simulink model "traj_rigid_body_example"  (R2018b)
settings: Solver=ode2  StartTime=0.0  StopTime=60  FixedStep=0.001  RelTol=1e-3
values from neighbouring files (symbols this model uses):
  cycle = true    [traj_controller_mass_point_example_init.m]    (also in traj_from_waypoints_example.m = false; traj_rigid_body_example_init.m)
  g = 9.81    [traj_controller_mass_point_example_init.m]    (also in traj_from_waypoints_example.m; traj_rigid_body_example_init.m)
  inital_point = waypoints(:,1)    [traj_controller_mass_point_example_init.m]    (also in traj_rigid_body_example_init.m)
  inital_vel_vec = inital_velo * T    [traj_controller_mass_point_example_init.m]    (also in traj_rigid_body_example_init.m)
  traj = trajFromWaypoints(traj_empty, waypoints, degree, cycle)    [traj_controller_mass_point_example_init.m]    (also in traj_from_waypoints_example.m = trajFromWaypoints(traj, waypoints, degree, cycle); traj_rigid_body_example_init.m)
  waypoints = [1 -1 0.2; 2 0 0.1; 1 1 0; -1 -1 0; -2 0 0.1; -1 1 0.2]'*50    [traj_controller_mass_point_example_init.m]    (also in traj_from_waypoints_example.m = [1 1 1; 2 2 2; 3 3 3; 4 4 4]'; traj_rigid_body_example_init.m)
libraries: actuators_lib x8, traj_lib x3, axes_transformation_lib x3, flightgear_visualization_lib x1, sensors_lib x1, quatAttitudeController_lib x1, rigidBody_lib x1
settings Model: Creator=Fgücker  LastModifiedBy=yannic

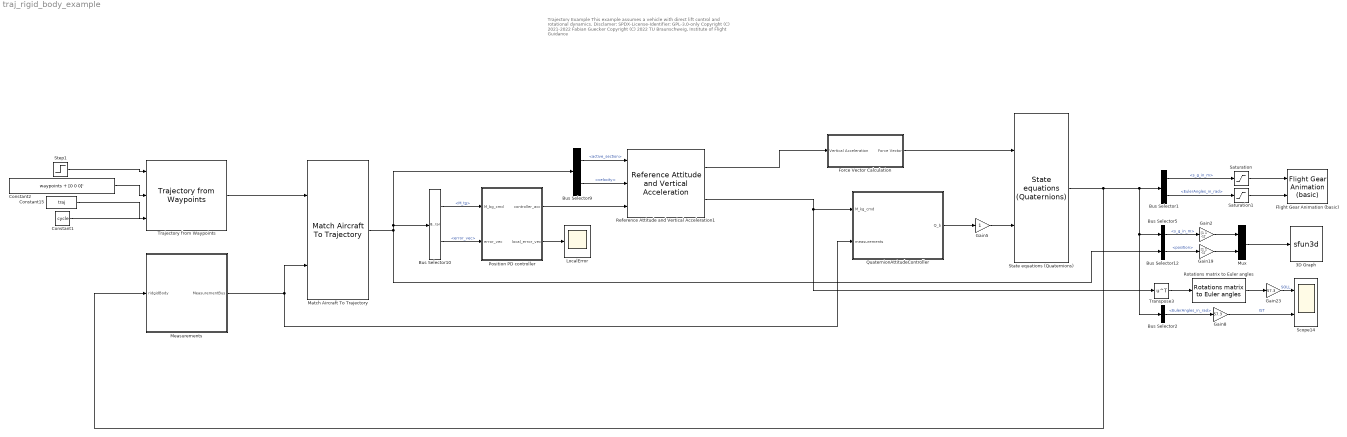
== system traj_rigid_body_example ==
  note: Trajectory Example
      |
      | This example assumes a vehicle with direct lift control and rotational dynamics.
      |
      | Disclamer:
      | SPDX-License-Identifier: GPL-3.0-only
      |
      | Copyright (C) 2021-2022 Fabian Guecker
      | Copyright (C) 2022 TU Braunschweig, Institute of Flight Guidance
  3D Graph : S-Function  LoadFcn=if exist('sfun3d','file'), sfun3d([],[],[],'LoadBlock'); end  FunctionName=sfun3d  Parameters=ax,T,np,cp,gd,ls,mk,mx,hd,tb  SFunctionDeploymentMode=off  EnableBusSupport=off  mask(3D Graph){np=2, ax=[-8 8 -8 8 -8 8]*20, mx=1e4, T=0.040, cp=[-1 -1 1]*50, gd=on, hd=off, tb=off, ls=-, mk=none}
      mask prompts: np "Number of moving points (lines)"; ax "Range: [xmin xmax  ymin ymax zmin zmax]"; mx "Max number of points in each line"; T "Sampling Time"; cp "Camera position (use [0 0 1] for 2D XY view)"; gd "Grid (on|off)"; hd "HeadMarkers (on|off)"; tb "Toolbar (on|off)"; ls "LineStyle"; mk "LineMarker"
      mask help:
      | This block plots the position of several points in the XYZ space. The input contains the coordinates of all the points (x1,y1,z1,x2,y2,z2,...).
      | The number of moving points (lines), the XYZ ranges, sampling time, camera position, and grid (among other things) can be set as mask parameters.
      settings: CopyFcn=if exist('sfun3d','file'), sfun3d([],[],[],'CopyBlock'); end  DeleteFcn=if exist('sfun3d','file'), sfun3d([],[],[],'DeleteBlock'); end  NameChangeFcn=if exist('sfun3d','file'), sfun3d([],[],[],'NameChange'); end
      mask Help:
      | This block plots the position of several points in the XYZ space. The input contains the coordinates of all the points (x1,y1,z1,x2,y2,z2,...).
      | The number of moving points (lines), the XYZ ranges, sampling time, camera position, and grid (among other things) can be set as mask parameters.
      mask TypeOptions ls: - | -- | : | -. | none
      mask TypeOptions mk: none | . | + | o | * | x | square | diamond | v | ^ | > | < | pentagram | hexagram
      mask Display: plot([.05 .95 .95 .05 .05],[.45 .45 .95 .95 .45], 0.5+cos(0:0.1:2*pi)*0.3,0.7+sin(0:0.1:2*pi)*0.2)
  Bus Selector1 : BusSelector  OutputSignals=s_g_in_m,EulerAngles_in_rad
  Bus Selector10 : BusSelector  OutputSignals=M_tg,error_vec
  Bus Selector12 : BusSelector  OutputSignals=position
  Bus Selector2 : BusSelector  OutputSignals=EulerAngles_in_rad
  Bus Selector5 : BusSelector  OutputSignals=s_g_in_m
  Bus Selector9 : BusSelector  OutputSignals=active_section,velocity
  Constant1 : Constant  Value=cycle  OutDataTypeStr=boolean
  Constant15 : Constant  Value=traj  OutDataTypeStr=Bus: trajectoryBus
  Constant2 : Constant  Value=waypoints + [0 0 0]'
  Flight Gear Animation (basic) : flightgear_visualization_lib/Flight Gear Animation (basic)  inital_lat=63.985024  inital_long=-22.597652  inital_height=70  remoteURL='127.0.0.1'  remotePort=5502
      settings: SourceProductName=LADAC
  Force Vector Calculation : Subsystem  mask{m=1}
      mask prompts: m "Mass of the aircraft"
  Gain19 : Gain  Gain=[1 1 -1]'
  Gain2 : Gain  Gain=[1 1 -1]'
  Gain23 : Gain  Gain=57.3
  Gain5 : Gain
  Gain8 : Gain  Gain=57.3
  LocalError : Scope
  Match Aircraft To Trajectory : traj_lib/Match Aircraft To Trajectory
      settings: SourceProductName=LADAC
  Measurements : Subsystem  mask{omega0=100, D=1}
      mask prompts: omega0 "Omega - Filter"; D "Damping D - Filter"
  Mux : Mux  Inputs=2
  Position PD controller : Subsystem
  QuaternionAttitudeController : Subsystem
  Reference Attitude and Vertical Acceleration1 : traj_lib/Reference Attitude and Vertical Acceleration  G0=9.81
      settings: SourceProductName=LADAC
  Rotations matrix to Euler angles : axes_transformation_lib/Rotations matrix to Euler angles  SystemSampleTime=-1
      settings: SourceProductName=LADAC
  Saturation : Saturate  UpperLimit=5000  LowerLimit=-5000
  Saturation1 : Saturate  UpperLimit=100*pi  LowerLimit=-100*pi
  Scope14 : Scope  NumInputPorts=2
  State equations (Quaternions) : rigidBody_lib/State equations (Quaternions)  m=1  I=eye(3)  g=9.81  omega_Kb_0=[0,0,0]'  q_bg_0=inital_quaternion'  V_Kb_0=[norm(inital_vel_vec);0;0]  s_g_0=inital_point+[0 0 0]'
  Step1 : Step  Time=0  SampleTime=0
  Trajectory from Waypoints : traj_lib/Trajectory from Waypoints  traj_params=traj_params
      settings: SourceProductName=LADAC
  Transpose3 : Math  Operator=transpose  SaturateOnIntegerOverflow=on
  wires:
  Bus Selector1/2 -> Saturation1/1  "<EulerAngles_in_rad>"
  Bus Selector1/1 -> Saturation/1  "<s_g_in_m>"
  QuaternionAttitudeController/1(Q_b) -> Gain5/1
  Bus Selector2/1 -> Gain8/1  "<EulerAngles_in_rad>"
  Bus Selector5/1 -> Gain2/1  "<s_g_in_m>"
  State equations (Quaternions)/1 -> Measurements/1(ridgidBody), Bus Selector5/1, Bus Selector2/1, Bus Selector1/1
  Saturation/1 -> Flight Gear Animation (basic)/1
  Saturation1/1 -> Flight Gear Animation (basic)/2
  Gain5/1 -> State equations (Quaternions)/2
  Gain2/1 -> Mux/1
  Mux/1 -> 3D Graph/1
  Gain19/1 -> Mux/2
  Gain23/1 -> Scope14/1  "SOLL"
  Measurements/1(MeasurementBus) -> Match Aircraft To Trajectory/2, QuaternionAttitudeController/2(measurements)
  Match Aircraft To Trajectory/1 -> Bus Selector9/1, Bus Selector10/1, Bus Selector12/1
  Bus Selector9/1 -> Reference Attitude and Vertical Acceleration1/1  "<active_section>"
  Bus Selector9/2 -> Reference Attitude and Vertical Acceleration1/2  "<velocity>"
  Bus Selector12/1 -> Gain19/1  "<position>"
  Constant1/1 -> ?
  Step1/1 -> Trajectory from Waypoints/1
  Constant15/1 -> Trajectory from Waypoints/3
  Constant2/1 -> Trajectory from Waypoints/2
  Position PD controller/1(controller_acc) -> Reference Attitude and Vertical Acceleration1/3
  Position PD controller/2(local_error_vec) -> LocalError/1
  Gain8/1 -> Scope14/2  "IST"
  Rotations matrix to Euler angles/1 -> Gain23/1
  Transpose3/1 -> Rotations matrix to Euler angles/1
  Reference Attitude and Vertical Acceleration1/2 -> Transpose3/1, QuaternionAttitudeController/1(M_kg_cmd)
  Bus Selector10/1 -> Position PD controller/1(M_bg_cmd)  "<M_tg>"
  Bus Selector10/2 -> Position PD controller/2(error_vec)  "<error_vec>"
  Reference Attitude and Vertical Acceleration1/1 -> Force Vector Calculation/1(Vertical Acceleration)
  Force Vector Calculation/1(Force Vector) -> State equations (Quaternions)/1
  Trajectory from Waypoints/1 -> Match Aircraft To Trajectory/1

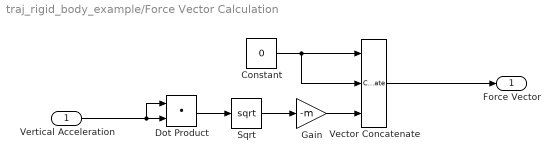
== system traj_rigid_body_example/Force Vector Calculation ==
  Vertical Acceleration : Inport
  Constant : Constant  Value=0
  Dot Product : DotProduct  InputSameDT=on  OutDataTypeStr=Inherit: Inherit via internal rule
  Gain : Gain  Gain=-m
  Sqrt : Sqrt  SaturateOnIntegerOverflow=on
  Vector Concatenate : Concatenate  NumInputs=3
  Force Vector : Outport
  wires:
  Vertical Acceleration/1 -> Dot Product/1, Dot Product/2
  Constant/1 -> Vector Concatenate/2, Vector Concatenate/1
  Vector Concatenate/1 -> Force Vector/1
  Dot Product/1 -> Sqrt/1
  Sqrt/1 -> Gain/1
  Gain/1 -> Vector Concatenate/3

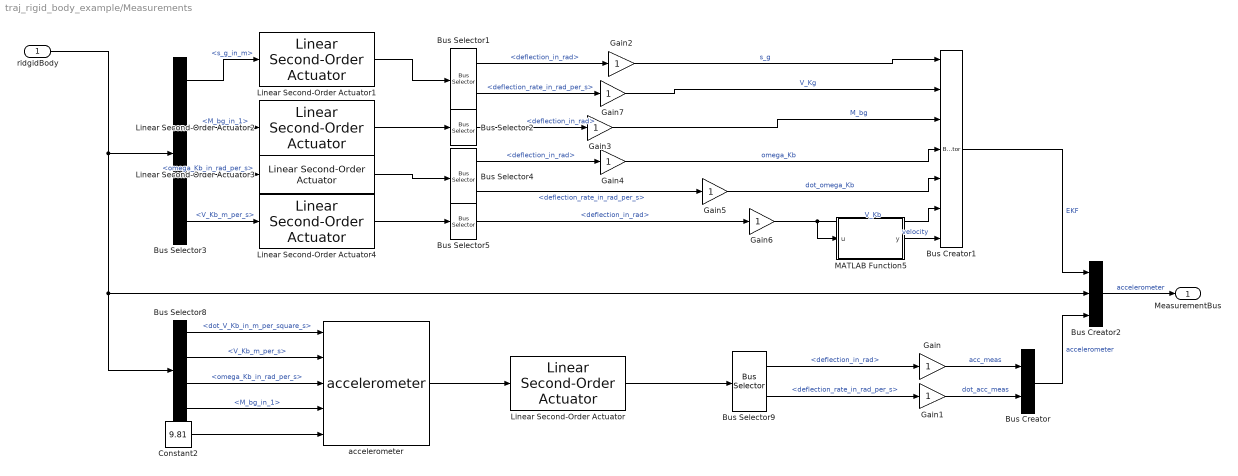
== system traj_rigid_body_example/Measurements ==
  ridgidBody : Inport
  Bus Creator : BusCreator  Inputs=2
  Bus Creator1 : BusCreator  Inputs=7
  Bus Creator2 : BusCreator  Inputs=3
  Bus Selector1 : BusSelector  OutputSignals=deflection_in_rad,deflection_rate_in_rad_per_s
  Bus Selector2 : BusSelector  OutputSignals=deflection_in_rad
  Bus Selector3 : BusSelector  OutputSignals=s_g_in_m,M_bg_in_1,omega_Kb_in_rad_per_s,V_Kb_m_per_s
  Bus Selector4 : BusSelector  OutputSignals=deflection_in_rad,deflection_rate_in_rad_per_s
  Bus Selector5 : BusSelector  OutputSignals=deflection_in_rad
  Bus Selector8 : BusSelector  OutputSignals=dot_V_Kb_in_m_per_square_s,V_Kb_m_per_s,omega_Kb_in_rad_per_s,M_bg_in_1
  Bus Selector9 : BusSelector  OutputSignals=deflection_in_rad,deflection_rate_in_rad_per_s
  Constant2 : Constant  Value=9.81
  Gain{,1..7} (8 alike) : Gain
  Linear Second-Order Actuator : actuators_lib/Linear Second-Order Actuator  omega=omega0  d=D  A_0=[0 0 -g]  dot_A_0=0
      settings: SourceProductName=LADAC
  Linear Second-Order Actuator{1..4} (4 alike) : actuators_lib/Linear Second-Order Actuator  omega=omega0  d=D  A_0=0  dot_A_0=0
      settings: SourceProductName=LADAC
  MATLAB Function5 : MATLAB Function  TreatAsAtomicUnit=on
  accelerometer : sensors_lib/accelerometer  SystemSampleTime=-1
      settings: SourceProductName=LADAC
  MeasurementBus : Outport
  wires:
  Bus Selector9/2 -> Gain1/1  "<deflection_rate_in_rad_per_s>"
  Bus Selector8/1 -> accelerometer/1  "<dot_V_Kb_in_m_per_square_s>"
  Linear Second-Order Actuator/1 -> Bus Selector9/1
  Bus Selector8/2 -> accelerometer/2  "<V_Kb_m_per_s>"
  Bus Selector8/3 -> accelerometer/3  "<omega_Kb_in_rad_per_s>"
  Constant2/1 -> accelerometer/5
  Bus Selector8/4 -> accelerometer/4  "<M_bg_in_1>"
  accelerometer/1 -> Linear Second-Order Actuator/1
  Bus Selector9/1 -> Gain/1  "<deflection_in_rad>"
  Gain/1 -> Bus Creator/1  "acc_meas"
  Gain1/1 -> Bus Creator/2  "dot_acc_meas"
  ridgidBody/1 -> Bus Creator2/2, Bus Selector8/1, Bus Selector3/1
  Linear Second-Order Actuator1/1 -> Bus Selector1/1
  Bus Selector3/1 -> Linear Second-Order Actuator1/1  "<s_g_in_m>"
  Bus Creator1/1 -> Bus Creator2/1  "EKF"
  Bus Creator2/1 -> MeasurementBus/1  "accelerometer"
  Bus Selector1/1 -> Gain2/1  "<deflection_in_rad>"
  Bus Selector1/2 -> Gain7/1  "<deflection_rate_in_rad_per_s>"
  Gain2/1 -> Bus Creator1/1  "s_g"
  Bus Selector3/2 -> Linear Second-Order Actuator2/1  "<M_bg_in_1>"
  Bus Selector3/3 -> Linear Second-Order Actuator3/1  "<omega_Kb_in_rad_per_s>"
  Linear Second-Order Actuator2/1 -> Bus Selector2/1
  Linear Second-Order Actuator3/1 -> Bus Selector4/1
  Bus Selector4/2 -> Gain5/1  "<deflection_rate_in_rad_per_s>"
  Bus Selector4/1 -> Gain4/1  "<deflection_in_rad>"
  Bus Selector2/1 -> Gain3/1  "<deflection_in_rad>"
  Gain3/1 -> Bus Creator1/3  "M_bg"
  Gain4/1 -> Bus Creator1/4  "omega_Kb"
  Gain5/1 -> Bus Creator1/5  "dot_omega_Kb"
  Bus Selector3/4 -> Linear Second-Order Actuator4/1  "<V_Kb_m_per_s>"
  Linear Second-Order Actuator4/1 -> Bus Selector5/1
  Bus Selector5/1 -> Gain6/1  "<deflection_in_rad>"
  Gain6/1 -> MATLAB Function5/1(u), Bus Creator1/6  "V_Kb"
  Gain7/1 -> Bus Creator1/2  "V_Kg"
  MATLAB Function5/1(y) -> Bus Creator1/7  "velocity"
  Bus Creator/1 -> Bus Creator2/3  "accelerometer"

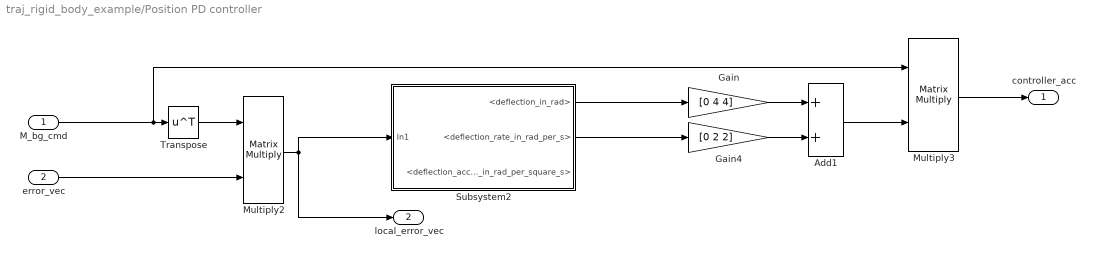
== system traj_rigid_body_example/Position PD controller ==
  M_bg_cmd : Inport
  error_vec : Inport  Port=2
  Add1 : Sum
  Gain : Gain  Gain=[0 4 4]
  Gain4 : Gain  Gain=[0 2 2]
  Multiply2 : Product  Multiplication=Matrix(*)
  Multiply3 : Product  Multiplication=Matrix(*)
  Subsystem2 : Subsystem
  Transpose : Math  Operator=transpose  SaturateOnIntegerOverflow=on
  controller_acc : Outport
  local_error_vec : Outport  Port=2
  wires:
  Gain4/1 -> Add1/2
  error_vec/1 -> Multiply2/2
  Gain/1 -> Add1/1
  Add1/1 -> Multiply3/2
  Transpose/1 -> Multiply2/1
  M_bg_cmd/1 -> Multiply3/1, Transpose/1
  Multiply3/1 -> controller_acc/1
  Multiply2/1 -> Subsystem2/1(In1), local_error_vec/1
  Subsystem2/1(<deflection_in_rad>) -> Gain/1
  Subsystem2/2(<deflection_rate_in_rad_per_s>) -> Gain4/1

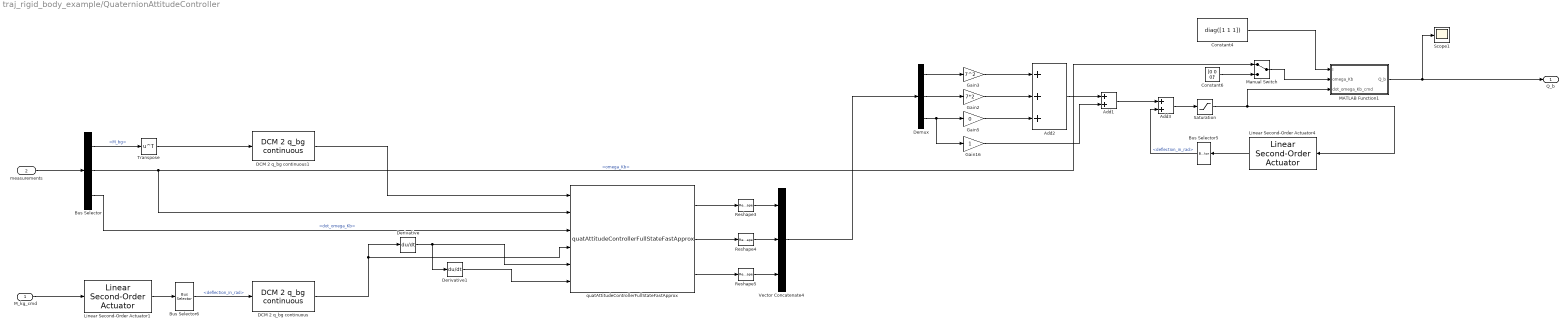
== system traj_rigid_body_example/QuaternionAttitudeController ==
  M_kg_cmd : Inport
  measurements : Inport  Port=2
  Add1 : Sum
  Add2 : Sum  Inputs=+++
  Add3 : Sum
  Bus Selector : BusSelector  OutputSignals=EKF.M_bg,EKF.omega_Kb,EKF.dot_omega_Kb
  Bus Selector5 : BusSelector  OutputSignals=deflection_in_rad
  Bus Selector6 : BusSelector  OutputSignals=deflection_in_rad
  Constant4 : Constant  Value=diag([1 1 1])  VectorParams1D=off
  Constant6 : Constant  Value=[0 0 0]'  VectorParams1D=off
  DCM 2 q_bg continuous : axes_transformation_lib/DCM 2 q_bg continuous
      settings: SourceProductName=LADAC
  DCM 2 q_bg continuous1 : axes_transformation_lib/DCM 2 q_bg continuous
      settings: SourceProductName=LADAC
  Demux : Demux  Outputs=3
  Derivative : Derivative
  Derivative1 : Derivative
  Gain16 : Gain
  Gain2 : Gain  Gain=7*2
  Gain3 : Gain  Gain=7^2
  Gain5 : Gain  Gain=0
  Linear Second-Order Actuator1 : actuators_lib/Linear Second-Order Actuator  omega=60  d=1  A_0=0  dot_A_0=0  start_steady_state=off
      settings: SourceProductName=LADAC
  Linear Second-Order Actuator4 : actuators_lib/Linear Second-Order Actuator  omega=80  d=1  A_0=[0 0 0]'  dot_A_0=0  start_steady_state=off
      settings: SourceProductName=LADAC
  MATLAB Function1 : MATLAB Function  TreatAsAtomicUnit=on
  Manual Switch : ManualSwitch
  Reshape3 : Reshape  OutputDimensionality=Column vector (2-D)
  Reshape4 : Reshape  OutputDimensionality=Column vector (2-D)
  Reshape5 : Reshape  OutputDimensionality=Column vector (2-D)
  Saturation : Saturate  UpperLimit=10  LowerLimit=-10
  Scope1 : Scope
  Transpose : Math  Operator=transpose  SaturateOnIntegerOverflow=on
  Vector Concatenate4 : Concatenate  NumInputs=3
  quatAttitudeControllerFullStateFastApprox : quatAttitudeController_lib/quatAttitudeControllerFullStateFastApprox  SystemSampleTime=-1
      settings: SourceProductName=LADAC
  Q_b : Outport
  wires:
  Bus Selector/3 -> quatAttitudeControllerFullStateFastApprox/3  "<dot_omega_Kb>"
  Derivative1/1 -> quatAttitudeControllerFullStateFastApprox/6
  Linear Second-Order Actuator1/1 -> Bus Selector6/1
  Vector Concatenate4/1 -> Demux/1
  Bus Selector6/1 -> DCM 2 q_bg continuous/1  "<deflection_in_rad>"
  Bus Selector/2 -> quatAttitudeControllerFullStateFastApprox/2, Manual Switch/1  "<omega_Kb>"
  Gain5/1 -> Add2/3
  DCM 2 q_bg continuous/1 -> quatAttitudeControllerFullStateFastApprox/4, Derivative/1
  Manual Switch/1 -> MATLAB Function1/2(omega_Kb)
  Add1/1 -> Add3/1
  Gain3/1 -> Add2/1
  Demux/2 -> Gain2/1
  Derivative/1 -> quatAttitudeControllerFullStateFastApprox/5, Derivative1/1
  M_kg_cmd/1 -> Linear Second-Order Actuator1/1
  Demux/1 -> Gain3/1
  Gain2/1 -> Add2/2
  Gain16/1 -> Add1/2
  Add2/1 -> Add1/1
  Constant6/1 -> Manual Switch/2
  Constant4/1 -> MATLAB Function1/1(I)
  Linear Second-Order Actuator4/1 -> Bus Selector5/1
  Demux/3 -> Gain5/1, Gain16/1
  measurements/1 -> Bus Selector/1
  MATLAB Function1/1(Q_b) -> Scope1/1, Q_b/1
  Add3/1 -> Saturation/1
  Bus Selector5/1 -> Add3/2  "<deflection_in_rad>"
  Saturation/1 -> Linear Second-Order Actuator4/1, MATLAB Function1/3(dot_omega_Kb_cmd)
  Bus Selector/1 -> Transpose/1  "<M_bg>"
  DCM 2 q_bg continuous1/1 -> quatAttitudeControllerFullStateFastApprox/1
  Transpose/1 -> DCM 2 q_bg continuous1/1
  quatAttitudeControllerFullStateFastApprox/1 -> Reshape3/1
  Reshape3/1 -> Vector Concatenate4/1
  Reshape4/1 -> Vector Concatenate4/2
  Reshape5/1 -> Vector Concatenate4/3
  quatAttitudeControllerFullStateFastApprox/2 -> Reshape4/1
  quatAttitudeControllerFullStateFastApprox/3 -> Reshape5/1

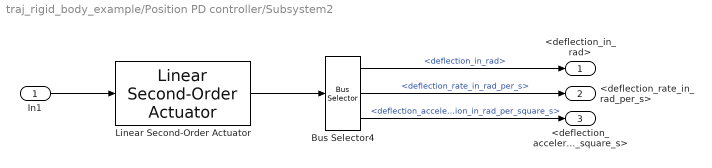
== system traj_rigid_body_example/Position PD controller/Subsystem2 ==
  In1 : Inport
  Bus Selector4 : BusSelector  OutputSignals=deflection_in_rad,deflection_rate_in_rad_per_s,deflection_acceleration_in_rad_per_square_s
  Linear Second-Order Actuator : actuators_lib/Linear Second-Order Actuator  omega=40  d=1  A_0=0  dot_A_0=0
      settings: SourceProductName=LADAC
  <deflection_in_rad> : Outport
  <deflection_rate_in_rad_per_s> : Outport  Port=2
  <deflection_acceleration_in_rad_per_square_s> : Outport  Port=3
  wires:
  Bus Selector4/2 -> <deflection_rate_in_rad_per_s>/1  "<deflection_rate_in_rad_per_s>"
  Bus Selector4/1 -> <deflection_in_rad>/1  "<deflection_in_rad>"
  Linear Second-Order Actuator/1 -> Bus Selector4/1
  Bus Selector4/3 -> <deflection_acceleration_in_rad_per_square_s>/1  "<deflection_acceleration_in_rad_per_square_s>"
  In1/1 -> Linear Second-Order Actuator/1

== matlab function traj_rigid_body_example/Measurements/MATLAB Function5 ==
  data: u input; y output
function y = fcn(u)

y = norm(u);

== matlab function traj_rigid_body_example/QuaternionAttitudeController/MATLAB Function1 ==
  data: I input; Q_b output; omega_Kb input; dot_omega_Kb_cmd input
function Q_b = fcn(I,omega_Kb,dot_omega_Kb_cmd)

Q_b = I * dot_omega_Kb_cmd + cross( omega_Kb, I * omega_Kb );

end
